simulink model "rc_circuit_diff_equ"  (R2026a)
settings: Solver=VariableStepAuto  StopTime=0.0001*5
settings Model: Creator=HAKAN SARI  LastModifiedBy=HAKAN SARI

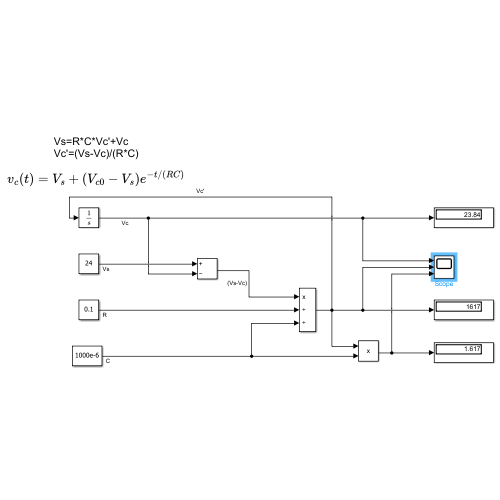
[thumbnail: Simulink's stored preview of the top-level diagram]
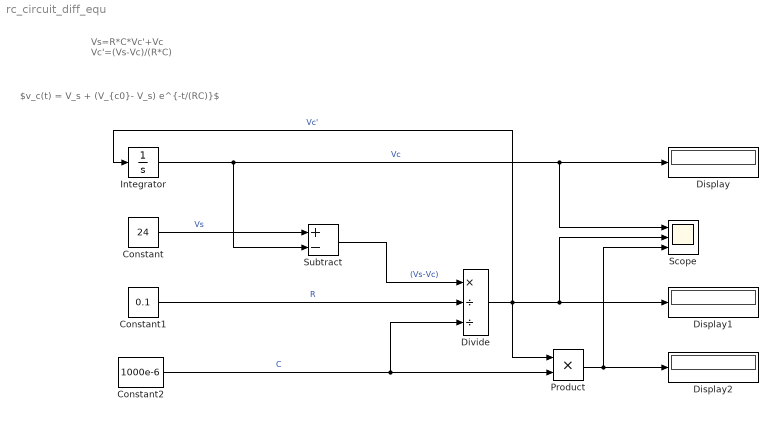
== system rc_circuit_diff_equ ==
  note: $v_c(t) = V_s + (V_{c0}- V_s) e^{-t/(RC)}$
  note: Vs=R*C*Vc'+Vc
      | Vc'=(Vs-Vc)/(R*C)
  Constant : Constant  Value=24
  Constant1 : Constant  Value=0.1
  Constant2 : Constant  Value=1000e-6
  Display : Display
  Display1 : Display
  Display2 : Display
  Divide : Product  Inputs=*//
  Integrator : Integrator
  Product : Product
  Scope : Scope  NumInputPorts=3
      settings: ActiveDisplayString=3  ActiveDisplayYMinimum=-28.180754280897403  ActiveDisplayYMaximum=269.79786158676637
  Subtract : Sum  Inputs=+-
  wires:
  Constant/1 -> Subtract/1  "Vs"
  Subtract/1 -> Divide/1  "(Vs-Vc)"
  Constant1/1 -> Divide/2  "R"
  Constant2/1 -> Divide/3, Product/2  "C"
  Divide/1 -> Product/1, Scope/2, Display1/1, Integrator/1  "Vc'"
  Integrator/1 -> Subtract/2, Scope/1, Display/1  "Vc"
  Product/1 -> Scope/3, Display2/1
